simulink model "Mission_C"  (R2023a)
settings: Solver=VariableStepAuto  StartTime=0.0  StopTime=10.0  RelTol=1e-3
settings Model: Creator=rose  LastModifiedBy=rose
settings OptimizationCC: DefaultParameterBehavior=Inlined

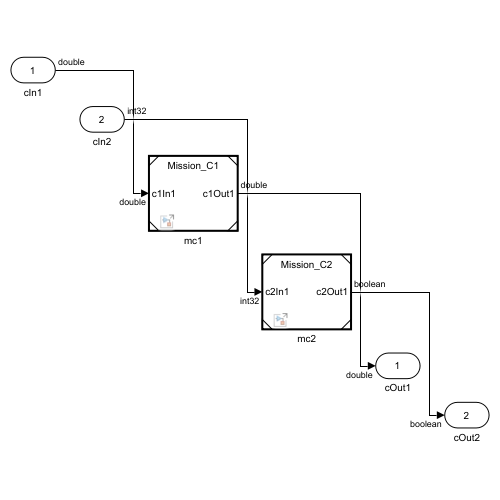
[thumbnail: Simulink's stored preview of the top-level diagram]
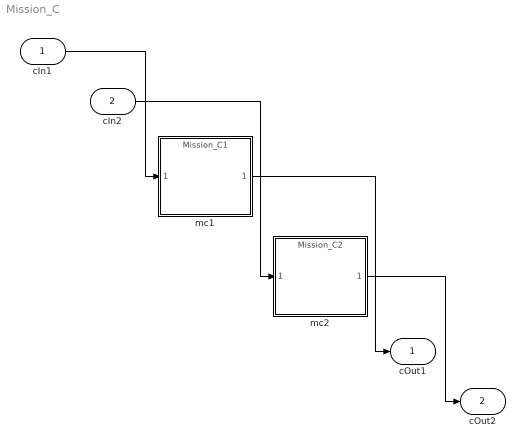
== system Mission_C ==
  cIn1 : Inport  OutDataTypeStr=double
  cIn2 : Inport  Port=2  OutDataTypeStr=int32
  mc1 : ModelReference  ModelNameDialog=Mission_C1  SimulationMode=Normal  ModelReferenceVersion=1.1
  mc2 : ModelReference  ModelNameDialog=Mission_C2  SimulationMode=Normal  ModelReferenceVersion=1.1
  cOut1 : Outport  OutDataTypeStr=double
  cOut2 : Outport  Port=2  OutDataTypeStr=boolean
  wires:
  cIn1/1 -> mc1/1
  cIn2/1 -> mc2/1
  mc1/1 -> cOut1/1
  mc2/1 -> cOut2/1
